simulink model "modele_chaine_codee"  (R2024b)
settings: Solver=FixedStepDiscrete  StartTime=0.0  StopTime=(Nsim-1)*Tb  FixedStep=Tec  RelTol=1e-3
values from neighbouring files (symbols this model uses):
  L = @(a, b) add_line(blk, a, b, 'autorouting', 'on')    [ajouter_codeur_registre.m]    (also in ajouter_decodeur_hamming.m; ajouter_modem_qpsk.m; ajouter_modem_qpsk_filtre.m; construire_modele_codeur_registre.m = @(a, b) add_line(mdl, a, b, 'autorouting', 'on'))
undefined symbols (not defined in the file or in its folder): Ac, dAlign, dPhase, graine, phaseC, sigma2e, Tb, Tc, Tec
settings Model: Creator=youka  LastModifiedBy=youka

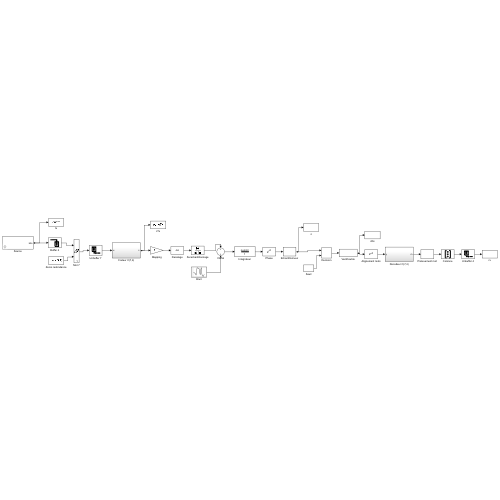
[thumbnail: Simulink's stored preview of the top-level diagram]
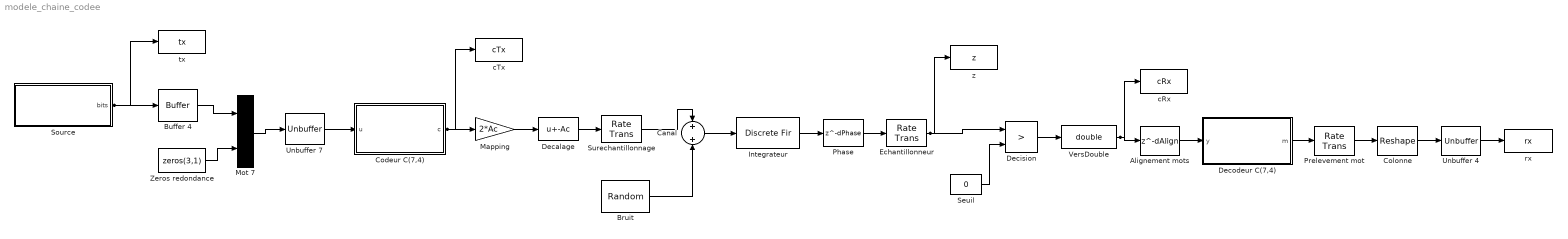
== system modele_chaine_codee ==
  Alignement mots : Delay  DelayLength=dAlign
  Bruit : RandomNumber  Variance=sigma2e  Seed=graine+1  SampleTime=Tec
  Buffer 4 : Buffer  N=4
  Canal : Sum
  Codeur C(7,4) : Subsystem
  Colonne : Reshape  OutputDimensionality=Column vector (2-D)
  Decalage : Bias  Bias=-Ac  SaturateOnIntegerOverflow=off
  Decision : RelationalOperator  Operator=>  OutDataTypeStr=boolean  RndMeth=Simplest  InputSameDT=off
  Decodeur C(7,4) : Subsystem
  Echantillonneur : RateTransition  OutPortSampleTime=Tc
  Integrateur : DiscreteFir  Coefficients=ones(1,L)/L
  Mapping : Gain  Gain=2*Ac
  Mot 7 : Concatenate  Mode=Multidimensional array
  Phase : Delay  DelayLength=dPhase
  Prelevement mot : RateTransition  OutPortSampleTime=4*Tb
  Seuil : Constant  Value=0  SampleTime=Tc
  Source : Subsystem  mask(Source binaire){p_m=0.5, Tb_m=Tb, graine_m=graine}
      mask prompts: p_m "Probabilité d'émettre un 1"; Tb_m "Durée d'un bit Tb (s)"; graine_m "Graine (Seed)"
      mask help: Source binaire sans mémoire : P(1) = p, un bit toutes les Tb secondes.
  Surechantillonnage : RateTransition  OutPortSampleTime=Tec
  Unbuffer 4 : Unbuffer
  Unbuffer 7 : Unbuffer
  VersDouble : DataTypeConversion  OutDataTypeStr=double  SaturateOnIntegerOverflow=off  RndMeth=Floor
  Zeros redondance : Constant  Value=zeros(3,1)  SampleTime=4*Tb
  cRx : ToWorkspace  VariableName=cRx  SampleTime=-1
  cTx : ToWorkspace  VariableName=cTx  SampleTime=-1
  rx : ToWorkspace  VariableName=rx  SampleTime=-1
  tx : ToWorkspace  VariableName=tx  SampleTime=-1
  z : ToWorkspace  VariableName=z  SampleTime=-1
  wires:
  Source/1(bits) -> tx/1, Buffer 4/1
  Buffer 4/1 -> Mot 7/1
  Zeros redondance/1 -> Mot 7/2
  Mot 7/1 -> Unbuffer 7/1
  Unbuffer 7/1 -> Codeur C(7,4)/1(u)
  Codeur C(7,4)/1(c) -> cTx/1, Mapping/1
  Mapping/1 -> Decalage/1
  Decalage/1 -> Surechantillonnage/1
  Surechantillonnage/1 -> Canal/1
  Bruit/1 -> Canal/2
  Canal/1 -> Integrateur/1
  Integrateur/1 -> Phase/1
  Phase/1 -> Echantillonneur/1
  Echantillonneur/1 -> z/1, Decision/1
  Seuil/1 -> Decision/2
  Decision/1 -> VersDouble/1
  VersDouble/1 -> cRx/1, Alignement mots/1
  Alignement mots/1 -> Decodeur C(7,4)/1(y)
  Decodeur C(7,4)/1(m) -> Prelevement mot/1
  Prelevement mot/1 -> Colonne/1
  Colonne/1 -> Unbuffer 4/1
  Unbuffer 4/1 -> rx/1

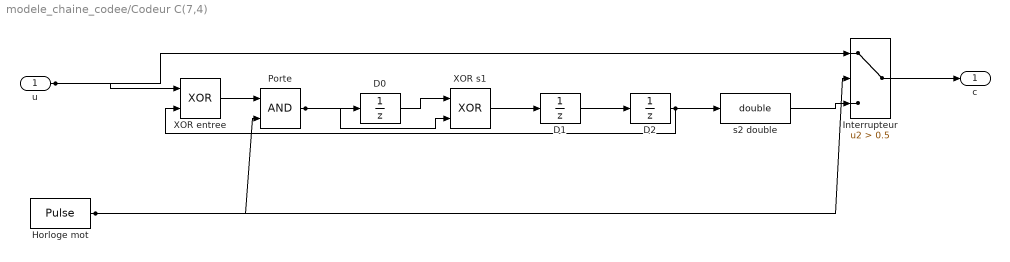
== system modele_chaine_codee/Codeur C(7,4) ==
  u : Inport
  D0 : UnitDelay  SampleTime=Tc  HasFrameUpgradeWarning=on
  D1 : UnitDelay  SampleTime=Tc  HasFrameUpgradeWarning=on
  D2 : UnitDelay  SampleTime=Tc  HasFrameUpgradeWarning=on
  Horloge mot : DiscretePulseGenerator  Period=7  PulseWidth=4  PhaseDelay=phaseC  SampleTime=Tc
  Interrupteur : Switch  Criteria=u2 > Threshold  Threshold=0.5  SaturateOnIntegerOverflow=off  InputSameDT=off
  Porte : Logic  AllPortsSameDT=off  OutDataTypeStr=boolean
  XOR entree : Logic  Operator=XOR  AllPortsSameDT=off  OutDataTypeStr=boolean
  XOR s1 : Logic  Operator=XOR  AllPortsSameDT=off  OutDataTypeStr=boolean
  s2 double : DataTypeConversion  OutDataTypeStr=double  SaturateOnIntegerOverflow=off  RndMeth=Floor
  c : Outport
  wires:
  u/1 -> XOR entree/1, Interrupteur/1
  D2/1 -> XOR entree/2, s2 double/1
  XOR entree/1 -> Porte/1
  Horloge mot/1 -> Porte/2, Interrupteur/2
  Porte/1 -> D0/1, XOR s1/2
  D0/1 -> XOR s1/1
  XOR s1/1 -> D1/1
  D1/1 -> D2/1
  s2 double/1 -> Interrupteur/3
  Interrupteur/1 -> c/1

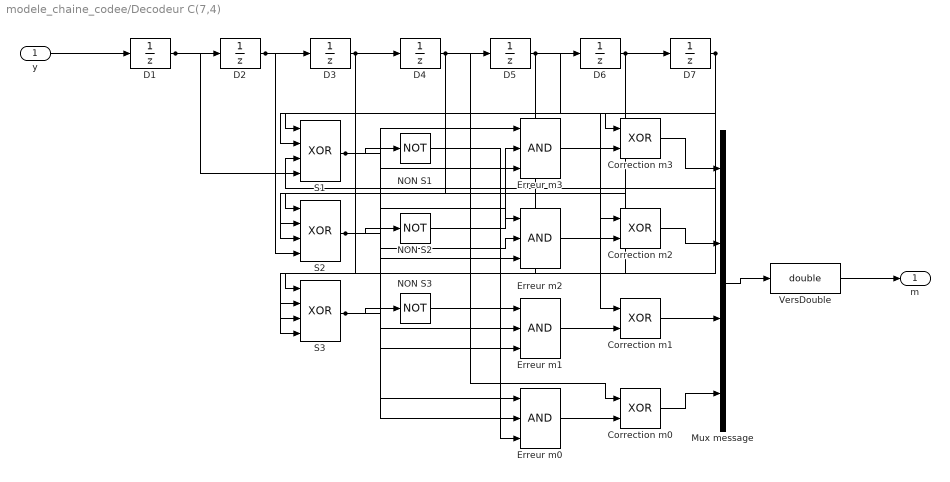
== system modele_chaine_codee/Decodeur C(7,4) ==
  y : Inport
  Correction m{0..3} (4 alike) : Logic  Operator=XOR  AllPortsSameDT=off  OutDataTypeStr=boolean
  D{1..7} (7 alike) : UnitDelay  SampleTime=Tc  HasFrameUpgradeWarning=on
  Erreur m{0..3} (4 alike) : Logic  Inputs=3  AllPortsSameDT=off  OutDataTypeStr=boolean
  Mux message : Mux
  NON S1 : Logic  Operator=NOT  AllPortsSameDT=off  OutDataTypeStr=boolean
  NON S2 : Logic  Operator=NOT  AllPortsSameDT=off  OutDataTypeStr=boolean
  NON S3 : Logic  Operator=NOT  AllPortsSameDT=off  OutDataTypeStr=boolean
  S1 : Logic  Operator=XOR  Inputs=4  AllPortsSameDT=off  OutDataTypeStr=boolean
  S2 : Logic  Operator=XOR  Inputs=4  AllPortsSameDT=off  OutDataTypeStr=boolean
  S3 : Logic  Operator=XOR  Inputs=4  AllPortsSameDT=off  OutDataTypeStr=boolean
  VersDouble : DataTypeConversion  OutDataTypeStr=double  SaturateOnIntegerOverflow=off  RndMeth=Floor
  m : Outport
  wires:
  y/1 -> D1/1
  D1/1 -> D2/1, S1/4
  D2/1 -> D3/1, S2/4
  D3/1 -> D4/1, S3/4
  D4/1 -> D5/1, S1/1, S2/1, Correction m0/1
  D5/1 -> D6/1, S2/2, S3/1, Correction m1/1
  D6/1 -> D7/1, S1/2, S2/3, S3/2, Correction m2/1
  D7/1 -> S1/3, S3/3, Correction m3/1
  S1/1 -> NON S1/1, Erreur m3/1, Erreur m2/1, Erreur m0/1
  S2/1 -> NON S2/1, Erreur m2/2, Erreur m1/2, Erreur m0/2
  S3/1 -> NON S3/1, Erreur m3/3, Erreur m2/3, Erreur m1/3
  NON S2/1 -> Erreur m3/2
  Erreur m3/1 -> Correction m3/2
  Erreur m2/1 -> Correction m2/2
  NON S1/1 -> Erreur m1/1
  Erreur m1/1 -> Correction m1/2
  NON S3/1 -> Erreur m0/3
  Erreur m0/1 -> Correction m0/2
  Correction m3/1 -> Mux message/1
  Correction m2/1 -> Mux message/2
  Correction m1/1 -> Mux message/3
  Correction m0/1 -> Mux message/4
  Mux message/1 -> VersDouble/1
  VersDouble/1 -> m/1

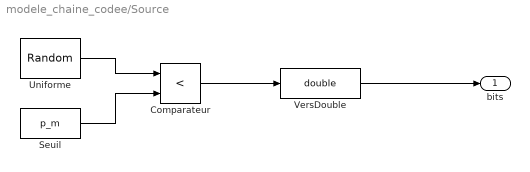
== system modele_chaine_codee/Source ==
  Comparateur : RelationalOperator  Operator=<  OutDataTypeStr=boolean  RndMeth=Simplest  InputSameDT=off
  Seuil : Constant  Value=p_m  SampleTime=Tb_m
  Uniforme : UniformRandomNumber  Minimum=0  Seed=graine_m  SampleTime=Tb_m
  VersDouble : DataTypeConversion  OutDataTypeStr=double  SaturateOnIntegerOverflow=off  RndMeth=Floor
  bits : Outport
  wires:
  Uniforme/1 -> Comparateur/1
  Seuil/1 -> Comparateur/2
  Comparateur/1 -> VersDouble/1
  VersDouble/1 -> bits/1
